simulink model "GHAME_Public"  (R2024a)
settings: Solver=ode8  StartTime=0.0  StopTime=Sim.simulation.duration  FixedStep=0.01  RelTol=1e-3
undefined symbols (not defined in the file): Data, DataPlant, IC, Sim, v0_BE_B
libraries: simulink_extras x8, simulink x1
(part 3 of 3)

== matlab function GHAME_Public/INS/INS/Inertial Navigation System ==
  settings: updateMethod=DISCRETE
  data: muc output; lonc output; latc output; psivdc output; thtvdc output; WBICB output; FSPCB output; dvbec output; SBII input; VBII input; TBI input; WBIB input; FSPB input; ZWG input; ZGPS input; ZST input; delta input; time input; alphacx output; betacx output; altc output; Sim parameter; nzc output; IC parameter; VBECB output; RICI output; EVBI output; ESBI output; MBC output; Data parameter; pdync output; GRAVG output; SBIIC output; VBECD output; TDCI output
function [muc, lonc, latc, psivdc, thtvdc, WBICB, FSPCB, dvbec, ...
    alphacx, betacx, altc, nzc, VBECB, RICI, EVBI, ESBI, MBC, pdync, ...
    GRAVG, SBIIC, VBECD, TDCI] = ins(SBII, VBII, TBI, WBIB, FSPB, ...
    ZWG, ZGPS, ZST, delta, time, Sim, IC, Data)
% INS  Inertial Navigation System model.
%
%   [muc, lonc, latc, psivdc, thtvdc, WBICB, FSPCB, dvbec, alphacx, ...
%       betacx, altc, nzc, VBECB, RICI, EVBI, ESBI, MBC, pdync, cmu, ...
%       c_CBF, dcda, GRAVG] = ins(vmass, SBII, VBII, TBI, WBIB, FSPB, ...
%       ZWG, ZGPS, ZST, delta, time, Sim, IC, Data)
%
%   Navigation states and derived flight quantities from the inertial
%   position, velocity, attitude, body rates and specific force. Based on
%   the CADAC++ 'ins' module of Zipfel, Modeling and Simulation of
%   Aerospace Vehicles.
%
%   Space stabilized INS error model. With Sim.mode.mINS = 1,
%   the tilt, velocity and position errors RICI, EVBI, ESBI are integrated
%   as discrete states with the trapezoidal rule. They start from init_ins
%   and are driven by
%     tilt rate      RICID = TBI' * EWBIB
%     vel err rate   EVBID = TICB*EFSPB - skew(RICI)*TICB*FSPCB + EGRAVI
%     pos err rate   ESBID = EVBI
%   With Sim.mode.mgps > 0 the GPS filter (gps_filter) estimates the
%   position and velocity errors at each GPS update, and they are removed
%   from ESBI and EVBI in the same step. With Sim.mode.mstar > 0 the star
%   tracker (startrack) measures the tilt at each star fix, and it is
%   removed from RICI before the velocity error is computed.
%
%   Onboard aerodynamic model (for rate_observer, with Sim.mode.mrateobs = 1)
%     MBC is the aerodynamic moment as the flight computer would compute
%     it, from the INS altitude, speed, alpha, beta and measured rates, a
%     US 1976 standard atmosphere and the aero tables. No wind is known
%     onboard, so the airspeed is taken as the INS Earth-relative speed.
%     cmu, c_CBF and dcda come from the same tables and are used by the
%     control allocation and the control barrier functions.
%
%   Simulink use (MATLAB Function block)
%     The block contains no random draws. All per run random values come
%     from Sim.ins, built with ins_setup(seed) before each run, and the
%     gyro random walk enters as the unit Gaussian input ZWG from a Random
%     Number block (mean 0, variance 1, sample time dt, seed per run).
%     The GPS Markov noises enter the same way as ZGPS, seed Sim.gps.seed_noise,
%     the star tracker noises as ZST, seed Sim.star.seed_noise.
%     The error states are persistent and reset at every simulation start.
%     The block must run with the discrete sample time dt = Sim.sample_time.
%
%   Inputs
%     vmass    [1x1]  Vehicle mass (kg)
%     SBII     [3x1]  Inertial position (m)
%     VBII     [3x1]  Inertial velocity (m/s)
%     TBI      [3x3]  Body wrt inertial transformation matrix (-)
%     WBIB     [3x1]  Inertial body rates in body axes (rad/s)
%     FSPB     [3x1]  Specific force in body axes (m/s^2)
%     ZWG      [3x1]  Unit Gaussian sample for the gyro random walk (-)
%     ZGPS     [9x1]  Unit Gaussian samples for the GPS Markov noises (-)
%     ZST      [6x1]  Unit Gaussian samples for the star tracker noises (-)
%     delta    [3x1]  Actuator positions [aileron; elevator; rudder] (rad)
%     time     [1x1]  Simulation time (s)
%     Sim      struct Earth model incl. GM, constants, INS mode mINS,
%                     GPS mode mgps, star tracker mode mstar, sample time,
%                     vehicle geometry, INS errors in Sim.ins (see
%                     ins_setup), GPS data in Sim.gps (see gps_setup),
%                     star tracker data in Sim.star (see startrack_setup)
%     IC       struct Earth rotation rate WEII3 (rad/s)
%     Data     struct Aero tables (Data.AeroCoefficients)
%
%   Outputs
%     muc      [1x1]  Aerodynamic roll angle (rad)
%     lonc     [1x1]  Longitude (rad)
%     latc     [1x1]  Geodetic latitude (rad)
%     psivdc   [1x1]  Heading angle (rad)
%     thtvdc   [1x1]  Flight path angle (rad)
%     WBICB    [3x1]  Measured body rates in body axes (rad/s)
%     FSPCB    [3x1]  Measured specific force in body axes (m/s^2)
%     dvbec    [1x1]  Earth-relative speed (m/s)
%     alphacx  [1x1]  Angle of attack (deg)
%     betacx   [1x1]  Angle of sideslip (deg)
%     altc     [1x1]  Altitude (m)
%     nzc      [1x1]  Normal load factor (-)
%     VBECB    [3x1]  Earth-relative velocity in body axes (m/s)
%     RICI     [3x1]  Tilt error (rad)
%     EVBI     [3x1]  Velocity error in inertial axes (m/s)
%     ESBI     [3x1]  Position error in inertial axes (m)
%     MBC      [3x1]  Onboard model of the aerodynamic moment, body axes (Nm)
%     pdync    [1x1]  Onboard dynamic pressure (Pa)
%     cmu      [3x3]  Moment control effectiveness, rows [roll; pitch; yaw],
%                     columns [aileron, elevator, rudder] (m)
%     c_CBF    [9x1]  Control barrier function terms, see cbf_terms
%     dcda     [1x2]  Slopes [dCD/dalpha, dCL/dalpha] (1/rad)
%     GRAVG    [3x1]  Gravitational acceleration, geocentric axes (m/s^2)
%
%   The diagnostics GPSDIAG (see gps_filter) and STDIAG (see startrack) are
%   computed below but are not part of the output list.
%
%   Author:    Thomas Harald Müller
%   GitHub:    https://github.com/ThomasHaraldMueller
%   Copyright: (c) 2026 Thomas Harald Müller, Hamburg, Germany
%   Free to use and modify, provided this notice is kept and the author is credited.

persistent RICI_s EVBI_s ESBI_s RICID EVBID ESBID

%% Constants and configuration
AGRAV    = Sim.earth.AGRAV;             % Standard gravity (m/s^2)
GM       = Sim.earth.GM;                % Earth gravitational constant (m^3/s^2)
GW_CLONG = Sim.earth.GW_CLONG;          % Greenwich longitude at the epoch (rad)
DEG      = Sim.constants.DEG;           % Radian to degree conversion (-)
PI       = Sim.constants.PI;
EPS      = Sim.constants.EPS;
WEII3    = IC.WEII3;                    % Earth rotation rate (rad/s)
mINS     = Sim.mode.mINS;               % INS mode, 0 = ideal INS
dt       = Sim.sample_time;             % Sample time (s)
E        = Sim.ins;                     % Sensor errors and initial error data

%% Error states at simulation start
if isempty(RICI_s)
    [ESBI_s, EVBI_s, RICI_s] = init_ins(mINS, E.frax, E.GAUSS0);
    RICID = zeros(3,1);
    EVBID = zeros(3,1);
    ESBID = zeros(3,1);
end

% GPS filter and star tracker diagnostics, filled in below
GPSDIAG = zeros(6,1);%#ok
STDIAG  = zeros(3,1);%#ok                                                       

%% Navigation solution
if mINS == 0
    % Ideal INS outputs
    TBIC  = TBI;
    FSPCB = FSPB;
    WBICB = WBIB;
    SBIIC = SBII;
    VBIIC = VBII;
else
    % INS derived position, needed for the gravity error
    SBIIC = ESBI_s + SBII;

    % Tilt error from the gyro errors
    [WBICB, EWBIB] = ins_gyro(WBIB, FSPB, ZWG, E, dt);
    RICID_NEW = TBI.' * EWBIB;
    RICI_s = RICI_s + dt/2 * (RICID_NEW + RICID);
    RICID  = RICID_NEW;
    TBIC   = TBI * (eye(3) - skew_sym(RICI_s));

    % Star tracker update of the tilt
    if Sim.mode.mstar > 0
        [URIC, upd_st, STDIAG] = startrack(TBI, TBIC, SBII, ZST, time, Sim); %#ok
        if upd_st
            RICI_s = RICI_s - URIC;
            TBIC   = TBI * (eye(3) - skew_sym(RICI_s));
        end
    end

    % Measured specific force
    EFSPB = ins_accl(FSPB, E);
    FSPCB = E.EWALKA + EFSPB + FSPB;

    % Velocity error from accelerometer, tilt and gravity errors
    EGRAVI    = ins_grav(ESBI_s, SBIIC, norm(SBII), GM);
    TICB      = TBIC.';
    EVBID_NEW = TICB * EFSPB - skew_sym(RICI_s) * TICB * FSPCB + EGRAVI;
    EVBI_s = EVBI_s + dt/2 * (EVBID_NEW + EVBID);
    EVBID  = EVBID_NEW;

    % Position error
    ESBID_NEW = EVBI_s;
    ESBI_s = ESBI_s + dt/2 * (ESBID_NEW + ESBID);
    ESBID  = ESBID_NEW;

    % INS derived position and velocity
    SBIIC = ESBI_s + SBII;
    VBIIC = EVBI_s + VBII;

    % GPS update of the position and velocity errors
    if Sim.mode.mgps > 0
        [SXH, VXH, upd, GPSDIAG] = gps_filter(SBII, VBII, SBIIC, VBIIC, ... 
                                              ZGPS, time, Sim); %#ok
        if upd
            ESBI_s = ESBI_s - SXH;
            EVBI_s = EVBI_s - VXH;
            SBIIC  = ESBI_s + SBII;
            VBIIC  = EVBI_s + VBII;
        end
    end
end

RICI = RICI_s;
EVBI = EVBI_s;
ESBI = ESBI_s;

%% Earth-relative velocity and incidence angles
VEIC  = [-WEII3 * SBIIC(2);
          WEII3 * SBIIC(1);
          0];
VBEIC = VBIIC - VEIC;
VBECB = TBIC * VBEIC;
dvbec = norm(VBECB);

alphac  = atan2(VBECB(3), VBECB(1));
betac   = asin(VBECB(2) / dvbec);
alphacx = alphac * DEG;
betacx  = betac  * DEG;

%% Geodetic position and attitude
[lonc, ~, latc, altc] = cad_geo84_in_cont(time, SBIIC, IC, Sim);
TDCI = cad_tdi84(lonc, latc, time, GW_CLONG, WEII3);

% Heading and flight path angle from the geodetic velocity
VBECD = TDCI * VBEIC;
if VBECD(1) == 0 && VBECD(2) == 0
    psivdc = 0;
    thtvdc = 0;
else
    psivdc = atan2(VBECD(2), VBECD(1));
    thtvdc = atan2(-VBECD(3), hypot(VBECD(1), VBECD(2)));
end

% Geodetic Euler angles
TBD = TBIC * TDCI.';
if abs(TBD(1,3)) < 1
    thtbdc = asin(-TBD(1,3));
    cthtbd = cos(thtbdc);
else
    thtbdc = sgn(-TBD(1,3)) * PI/2;
    cthtbd = EPS;                       % Prevents division by zero at +-90 deg
end
cpsi   = clamp_value(TBD(1,1) / cthtbd, -1, 1);
cphi   = clamp_value(TBD(3,3) / cthtbd, -1, 1);
psibdc = acos(cpsi) * sgn(TBD(1,2));                                        %#ok<NASGU>
phibdc = acos(cphi) * sgn(TBD(2,3));

% Aerodynamic roll angle
num = tan(phibdc) + tan(betac) * ...
      (tan(thtbdc) * cos(alphac) / cos(phibdc) - sin(alphac) / cos(thtbdc));
den = 1 + tan(thtbdc) * sin(alphac) / (cos(betac) * cos(phibdc));
muc = atan2(num, den);

% Normal load factor
nzc = -FSPCB(3) / AGRAV;

%% Air data from the standard atmosphere at the INS altitude
[rhoc, vsoundc] = atmosphere76(altc);
vmachc = dvbec / vsoundc;
pdync  = 0.5 * rhoc * dvbec^2;

GRAVG = cad_grav84(SBIIC, Sim);
%% Onboard aerodynamic model
G = Sim.vehicle.geometry;

% Earth-relative body rates in deg/s, as the aero tables expect them
WBECBx = (WBICB - TBIC * [0; 0; WEII3]) * DEG;

[c_mom] = aero_model(delta * DEG, vmachc, dvbec, alphacx, betacx, ...
                          WBECBx, Data.AeroCoefficients, Sim);
MBC = pdync * G.refa * [G.refb * c_mom(1);
                        G.refc * c_mom(2);
                        G.refb * c_mom(3)];
end


%% Local functions, INS sensor and error models =========================

function [WBICB, EWBIB] = ins_gyro(WBIB, FSPB, ZWG, E, dt)
% INS_GYRO  Gyro measured body rates and their error, with misalignment,
%   scale factor, bias, mass unbalance and random walk.

% Misalignment and scale factor plus bias
EGB   = diag(E.ESCALG) + skew_sym(E.EMISG);
EMSBG = E.EBIASG + EGB * WBIB;

% Spin axis sensitivity (mass unbalance)
EUG = E.EUNBG .* FSPB;

% Random walk, white noise with intensity EWALKG
EWG = E.EWALKG / sqrt(dt) * ZWG;

% Total error and measured body rates
EWBIB = EMSBG + EUG + EWG;
WBICB = WBIB + EWBIB;
end


function EFSPB = ins_accl(FSPB, E)
% INS_ACCL  Accelerometer error with misalignment, scale factor and bias.

EAB   = diag(E.ESCALA) + skew_sym(E.EMISA);
EFSPB = E.EBIASA + EAB * FSPB;
end


function EGRAVI = ins_grav(ESBI, SBIIC, dbi, GM)
% INS_GRAV  First order gravitational acceleration error (Zipfel, Eq. 10.94).

dbic   = norm(SBIIC);
ed     = dbic - dbi;
dum    = GM / dbic^3;
EGRAVI = -dum * ESBI - 3 * dum * ed / dbic * SBIIC;
end


%% Local functions, onboard aerodynamic model ===========================

function [alpha_vec, mach_vec, dalpha_deg] = aero_grid()
% AERO_GRID  Breakpoints of the aero tables and the step used for the
%   central differences in alpha.
%
%     alpha_vec   Angle of attack breakpoints (deg)
%     mach_vec    Mach number breakpoints (-)
%     dalpha_deg  Step of the central difference in alpha (deg)

alpha_vec  = (-3:3:+21);
mach_vec   = [0.4 0.6 0.8 0.9 0.95 1.05 1.2 1.5 2.0 3.0 6.0 12.0 24.0];
dalpha_deg = 1.0;
end


function c_mom = aero_model(deltax, vmach, DVBA, alphax, betax, WBEBx, Tab, Sim)
% AERO_MODEL  Onboard body-axis moment coefficients [Cl; Cm; Cn] and the
%   moment control effectiveness. Same tables and units as the plant
%   aerodynamics function, angles and deflections in deg, rates in deg/s.

RAD  = Sim.constants.RAD;
refb = Sim.vehicle.geometry.refb;
refc = Sim.vehicle.geometry.refc;
[alpha_vec, mach_vec] = aero_grid();

% Table lookup, clamped to the table range
vm = clamp_value(vmach,  mach_vec(1),  mach_vec(end));
al = clamp_value(alphax, alpha_vec(1), alpha_vec(end));
lk = @(table) interp2(mach_vec, alpha_vec, table, vm, al, 'linear');

% Nondimensional rates p*b/(2V), q*c/(2V), r*b/(2V)
pn = WBEBx(1) * RAD * refb / (2 * DVBA);
qn = WBEBx(2) * RAD * refc / (2 * DVBA);
rn = WBEBx(3) * RAD * refb / (2 * DVBA);

% Rolling, pitching and yawing moment
cll = lk(Tab.CLLB_tab) * betax + lk(Tab.CLLDA_tab) * deltax(1) + ...
      lk(Tab.CLLDR_tab) * deltax(3) + lk(Tab.CLLP_tab) * pn + lk(Tab.CLLR_tab) * rn;
clm = lk(Tab.CM0_tab) + lk(Tab.CMA_tab) * alphax + lk(Tab.CMDE_tab) * deltax(2) + ...
      lk(Tab.CMQ_tab) * qn;
cln = lk(Tab.CNB_tab) * betax + lk(Tab.CNDA_tab) * deltax(1) + ...
      lk(Tab.CNDR_tab) * deltax(3) + lk(Tab.CNP_tab) * pn + lk(Tab.CNR_tab) * rn;
c_mom = [cll; clm; cln];

end


%% Local functions, GPS =================================================

function [SXH, VXH, upd, GPSDIAG] = gps_filter(SBII, VBII, SBIIC, VBIIC, ZGPS, time, Sim)
% GPS_FILTER  GPS receiver and extended Kalman filter for INS aiding.
%
%   [SXH, VXH, upd, GPSDIAG] = gps_filter(SBII, VBII, SBIIC, VBIIC, ...
%       ZGPS, time, Sim)
%
%   Port of the CADAC++ 'gps' module of Zipfel, Modeling and Simulation of
%   Aerospace Vehicles. Four pseudo-ranges and four range rates are measured
%   from the four GPS satellites (quadriga) with the lowest GDOP. An 8 state
%   error filter (3 position, 3 velocity, user clock bias and frequency)
%   estimates the INS position and velocity errors at every GPS update.
%   The caller (ins) subtracts SXH and VXH from its error states when
%   upd = 1. The filter state is reset to zero after each update.
%
%   GPS is used in a run with Sim.mode.mgps = 1. Signal acquisition takes
%   Sim.gps.gps_acqtime before the first update. Internal GPS mode
%     0  no GPS
%     1  initialize filter, start signal acquisition
%     2  filter extrapolation between updates
%     3  update epoch, measurement and filter correction
%
%   Measurement errors are pseudo-range biases (constant per run), first
%   order Markov noise on pseudo-ranges, range rates and user clock
%   frequency, and the user clock bias obtained by integrating the clock
%   frequency error. The Markov processes are driven by the unit Gaussian
%   input ZGPS, which comes from a Random Number block in Simulink.
%
%   Inputs
%     SBII     [3x1]  True inertial position (m)
%     VBII     [3x1]  True inertial velocity (m/s)
%     SBIIC    [3x1]  INS inertial position (m)
%     VBIIC    [3x1]  INS inertial velocity (m/s)
%     ZGPS     [9x1]  Unit Gaussian samples for the Markov noises,
%                     [pseudo-range 1-4; range rate 1-4; clock frequency] (-)
%     time     [1x1]  Simulation time (s)
%     Sim      struct Earth model, sample time, GPS mode, GPS data in Sim.gps
%
%   Outputs
%     SXH      [3x1]  Estimated INS position error, inertial axes (m)
%     VXH      [3x1]  Estimated INS velocity error, inertial axes (m/s)
%     upd      [1x1]  1 at an update epoch, else 0 (-)
%     GPSDIAG  [6x1]  [std pos (m); std vel (m/s); std clock bias (m);
%                      GDOP (-); GPS mode (-); update flag (-)]
%
%   Author:    Thomas Harald Müller
%   GitHub:    https://github.com/ThomasHaraldMueller
%   Copyright: (c) 2026 Thomas Harald Müller, Hamburg, Germany
%   Free to use and modify, provided this notice is kept and the author is credited.

persistent mgps PP QQ RR PHI gps_epoch gps_acq ucbias_error ucfreqm XM gdop
persistent SV rsi wsi incl

G  = Sim.gps;
dt = Sim.sample_time;

% Initialization at simulation start
if isempty(mgps)
    mgps         = Sim.mode.mgps;       % 0: without GPS, 1: with GPS
    PP           = zeros(8);
    QQ           = zeros(8);
    RR           = zeros(8);
    PHI          = eye(8);
    gps_epoch    = 0;
    gps_acq      = 0;
    ucbias_error = G.ucbias0;           % User clock bias error (m)
    ucfreqm      = 0;                   % Clock frequency error, last step (m/s)
    XM           = G.markov0;           % Markov states [pr 1-4; dr 1-4; ucfreq]
    gdop         = 0;
    [SV, rsi, wsi, incl] = gps_sv_init(Sim.earth.GM);
end

SXH = zeros(3,1);
VXH = zeros(3,1);
upd = 0;

% First order Markov noises, exact discretization
a  = exp(-dt ./ G.tau_markov);
XM = a .* XM + G.sig_markov .* sqrt(1 - a.^2) .* ZGPS;
pr_noise     = XM(1:4);                 % Pseudo-range noise (m)
dr_noise     = XM(5:8);                 % Range rate noise (m/s)
ucfreq_error = XM(9);                   % User clock frequency error (m/s)

% Filter initialization, also used to re-acquire after a loss of satellites
if mgps == 1
    fp = 1 + G.factp;
    fq = 1 + G.factq;
    fr = 1 + G.factr;
    PP = diag(([G.ppos*[1 1 1], G.pvel*[1 1 1], G.pclockb, G.pclockf] * fp).^2);
    QQ = diag(([G.qpos*[1 1 1], G.qvel*[1 1 1], G.qclockb, G.qclockf] * fq).^2);
    RR = diag(([G.rpos*[1 1 1 1], G.rvel*[1 1 1 1]] * fr).^2);

    % Error dynamics and state transition matrix, constant
    FF = zeros(8);
    FF(1,4) = 1;
    FF(2,5) = 1;
    FF(3,6) = 1;
    FF(7,8) = 1;
    FF(8,8) = -1 / G.uctime_cor;
    PHI = eye(8) + FF * dt + FF * FF * (dt^2 / 2);

    gps_acq   = 1;
    gps_epoch = time;
    mgps      = 2;
end

% Clock error growth and covariance extrapolation
if mgps == 2
    if gps_acq
        dtime_gps = G.gps_acqtime;      % Signal acquisition delay (s)
    else
        dtime_gps = G.gps_step;         % Update interval (s)
    end
    if time - gps_epoch >= dtime_gps - 1e-9
        mgps = 3;
    end

    % User clock bias from the frequency error, trapezoidal integration
    ucbias_error = ucbias_error + (ucfreq_error + ucfreqm) * dt/2;
    ucfreqm      = ucfreq_error;

    PP = PHI * (PP + QQ * dt/2) * PHI.' + QQ * dt/2;
end

% Update epoch
if mgps == 3
    gps_acq   = 0;
    gps_epoch = time;
    [SSQ, VSQ, gdop_q, nvis] = gps_quadriga(SV, rsi, wsi, incl, ...
        G.almanac_time, G.del_rearth, Sim.earth.REARTH, time, SBII);

    if nvis < 4
        % Not enough satellites visible, re-acquire
        mgps = 1;
    else
        gdop = gdop_q;
        ZZ = zeros(8,1);
        HH = zeros(8,8);
        for i = 1:4
            SSII = SSQ(:,i);
            VSII = VSQ(:,i);

            % True and measured pseudo-range and range rate
            SSBI      = SSII - SBII;
            dsb       = norm(SSBI);
            USSBI     = SSBI / dsb;
            dsb_meas  = dsb + G.pr_bias(i) + pr_noise(i) + ucbias_error;
            dvsb      = (VSII - VBII).' * USSBI;
            dvsb_meas = dvsb + dr_noise(i) + ucfreq_error;

            % INS derived pseudo-range and range rate
            SSBIC = SSII - SBIIC;
            dsbc  = norm(SSBIC);
            dvsbc = (VSII - VBIIC).' * SSBIC / dsbc;

            % Measurement residuals and observation matrix
            ZZ(i)       = dsb_meas  - dsbc;
            ZZ(i+4)     = dvsb_meas - dvsbc;
            HH(i,1:3)   = USSBI.';
            HH(i,7)     = 1;
            HH(i+4,4:6) = USSBI.';      % Range rate residual in m/s, no
            HH(i+4,8)   = 1;            % gps_step factor (C++ used one)
        end

        % Kalman gain, state and covariance correction
        KK = (PP * HH.') / (HH * PP * HH.' + RR);
        XH = KK * ZZ;
        PP = (eye(8) - KK * HH) * PP;
        PP = (PP + PP.') / 2;

        % User clock bias correction
        ucbias_error = ucbias_error - XH(7);

        % Estimated INS errors, handed to ins
        SXH  = XH(1:3);
        VXH  = XH(4:6);
        upd  = 1;
        mgps = 2;
    end
end

GPSDIAG = [sqrt(PP(1,1)); sqrt(PP(4,4)); sqrt(PP(7,7)); gdop; mgps; upd];
end


function [SSQ, VSQ, gdop, nvis] = gps_quadriga(SV, rsi, wsi, incl, almanac_time, del_rearth, REARTH, time, SBII)
% GPS_QUADRIGA  Visible GPS satellites and the four with the lowest GDOP.
%   Circular orbits, 6 planes at 60 deg right ascension spacing, 55 deg
%   inclination. Returns their inertial positions and velocities as
%   columns, nvis < 4 means no valid quadriga.

% Satellite positions and velocities, argument of latitude propagated in time
Om  = SV(:,1);
u   = SV(:,2) + (almanac_time + time) * wsi;
si  = sin(incl);
ci  = cos(incl);
vel = rsi * wsi;

SSII = rsi * [ (cos(Om).*cos(u) - sin(Om).*sin(u)*ci).';
               (sin(Om).*cos(u) + cos(Om).*sin(u)*ci).';
               (sin(u)*si).' ];
VSII = vel * [ (-cos(Om).*sin(u) - sin(Om).*cos(u)*ci).';
               (-sin(Om).*sin(u) + cos(Om).*cos(u)*ci).';
               (cos(u)*si).' ];

% Visibility, inside the cone of the satellite or high enough for line of sight
dbi     = norm(SBII);
rclear  = REARTH + del_rearth;          % Radius for clear signal reception (m)
epsilon = acos(rclear / rsi);           % Grazing angle at the Earth center (rad)

vis  = zeros(24,1);
nvis = 0;
for i = 1:24
    cdel  = SSII(:,i).' * SBII / (rsi * dbi);
    delta = acos(clamp_value(cdel, -1, 1));
    rmin  = rclear / cos(delta - epsilon);
    if delta < epsilon || (rmin > 0 && rmin < dbi)
        nvis = nvis + 1;
        vis(nvis) = i;
    end
end

SSQ  = zeros(3,4);
VSQ  = zeros(3,4);
gdop = 1e10;
if nvis < 4
    return;
end

% Quadriga with the lowest GDOP among all combinations of visible satellites
quad = vis(1:4);
for i1 = 1:nvis-3
    for i2 = i1+1:nvis-2
        for i3 = i2+1:nvis-1
            for i4 = i3+1:nvis
                s = [vis(i1); vis(i2); vis(i3); vis(i4)];
                HGPS = ones(4,4);
                for m = 1:4
                    d = SBII - SSII(:,s(m));
                    HGPS(m,1:3) = d.' / norm(d);
                end
                M = HGPS * HGPS.';
                if rcond(M) > 1e-12
                    gdop_local = sqrt(trace(inv(M)));
                    if gdop_local < gdop
                        gdop = gdop_local;
                        quad = s;
                    end
                end
            end
        end
    end
end

SSQ = SSII(:,quad);
VSQ = VSII(:,quad);
end


function [SV, rsi, wsi, incl] = gps_sv_init(GM)
% GPS_SV_INIT  GPS constellation from the week 224 almanac (2003),
%   reduced to circular orbits. Rows are slots 1-24, planes A-F with four
%   satellites each, [right ascension (rad), argument of latitude (rad)].

SV = [ 0.9947,  1.0371;   % A plane
       0.9947,  2.7284;
       0.9947, -2.9855;
       0.9947, -0.9112;
       1.9197,  1.6417;   % B plane
       1.9197, -2.2572;
       1.9197, -0.7270;
       1.9197, -0.1626;
       2.9668,  0.5080;   % C plane
       2.9668,  2.1743;
       2.9668,  2.7649;
       2.9668, -1.8197;
       4.0140,  0.9408;   % D plane
       4.0140,  2.4279;
       4.0140, -3.1153;
       4.0140, -0.7710;
       5.0611,  1.3270;   % E plane
       5.0611,  2.1057;
       5.0611, -2.5338;
       5.0611, -0.2883;
       6.1082,  0.3998;   % F plane
       6.1082,  2.3427;
       6.1082, -1.8972;
       6.1082, -1.4035 ];

rsi  = 26560000;                        % Orbit radius (m)
wsi  = sqrt(GM / rsi^3);                % Orbital rate, half a sidereal day (rad/s)
incl = 0.95986;                         % Inclination, 55 deg (rad)
end


%% Local functions, star tracker ========================================

function [URIC, upd, STDIAG] = startrack(TBI, TBIC, SBII, ZST, time, Sim)
% STARTRACK  Star tracker for INS tilt correction.
%
%   [URIC, upd, STDIAG] = startrack(TBI, TBIC, SBII, ZST, time, Sim)
%
%   Port of the CADAC++ 'startrack' module of Zipfel, Modeling and
%   Simulation of Aerospace Vehicles. From a catalog of 25 bright stars the
%   visible ones are selected and the three with the largest parallelepiped
%   volume (triad) are tracked. Each star direction is measured in body
%   axes with the true attitude, corrupted by tracker bias and noise, and
%   converted back to inertial axes with the INS attitude TBIC. Comparing
%   measured and true directions gives I + skew(RICI), from which the INS
%   tilt is read directly. The caller (ins) subtracts URIC from RICI when
%   upd = 1. There is no filter, every fix replaces the tilt estimate.
%
%   The star tracker is used in a run with Sim.mode.mstar = 1. It works only
%   above Sim.star.startrack_alt, acquisition takes Sim.star.star_acqtime
%   before the first fix. Internal mode
%     0  no star tracker
%     1  initialized, waiting for the minimum altitude
%     2  waiting for the next fix
%     3  star fix and tilt correction
%
%   Inputs
%     TBI      [3x3]  True body wrt inertial transformation matrix (-)
%     TBIC     [3x3]  INS body wrt inertial transformation matrix (-)
%     SBII     [3x1]  True inertial position (m)
%     ZST      [6x1]  Unit Gaussian samples for the Markov noises,
%                     [azimuth 1-3; elevation 1-3] (-)
%     time     [1x1]  Simulation time (s)
%     Sim      struct Earth model, sample time, star tracker mode, data in
%                     Sim.star (see startrack_setup)
%
%   Outputs
%     URIC     [3x1]  Measured INS tilt, inertial axes (rad)
%     upd      [1x1]  1 at a star fix, else 0 (-)
%     STDIAG   [3x1]  [triad volume (-); star tracker mode (-); update flag (-)]
%
%   Author:    Thomas Harald Müller
%   GitHub:    https://github.com/ThomasHaraldMueller
%   Copyright: (c) 2026 Thomas Harald Müller, Hamburg, Germany
%   Free to use and modify, provided this notice is kept and the author is credited.

persistent mstar starfix_epoch star_acq XM star_volume

S  = Sim.star;
dt = Sim.sample_time;

% Initialization at simulation start
if isempty(mstar)
    mstar         = Sim.mode.mstar;     % 0: without star tracker, 1: with
    starfix_epoch = 0;
    star_acq      = 0;
    XM            = S.markov0;          % Markov states [az 1-3; el 1-3]
    star_volume   = 0;
end

URIC = zeros(3,1);
upd  = 0;

% First order Markov noises, exact discretization
a  = exp(-dt ./ S.tau_markov);
XM = a .* XM + S.sig_markov .* sqrt(1 - a.^2) .* ZST;

% Altitude over the mean Earth radius, only used for the availability check
alt = norm(SBII) - Sim.earth.REARTH;

% Initialization, acquisition starts once above the dense atmosphere
if mstar == 1
    star_acq      = 1;
    starfix_epoch = time;
    if alt > S.startrack_alt
        mstar = 2;
    end
end

% Delay before the first fix and between fixes
if mstar == 2
    if star_acq
        dtime_star = S.star_acqtime;    % Initial acquisition delay (s)
    else
        dtime_star = S.star_step;       % Fix interval (s)
    end
    if time - starfix_epoch >= dtime_star - 1e-9 && alt > S.startrack_alt
        mstar = 3;
    end
end

% Star fix
if mstar == 3
    star_acq      = 0;
    starfix_epoch = time;
    mstar         = 2;
    [UTRIAD, vol, nvis] = star_triad(star_catalog(), S.star_el_min * pi/180, SBII);

    if nvis >= 3
        star_volume = vol;
        TRIAD_MEAS  = zeros(3,3);
        for i = 1:3
            % True direction in body axes, azimuth and elevation
            USIB = TBI * UTRIAD(:,i);
            az   = atan2(USIB(2), USIB(1));
            el   = atan2(-USIB(3), hypot(USIB(1), USIB(2)));

            % Measurement with tracker bias and noise
            az_m  = az + S.az_bias(i) + XM(i);
            el_m  = el + S.el_bias(i) + XM(i+3);
            USIBM = [cos(el_m) * cos(az_m);
                     cos(el_m) * sin(az_m);
                    -sin(el_m)];

            % Back to inertial axes with the INS attitude, the tilt enters here
            TRIAD_MEAS(:,i) = TBIC.' * USIBM;
        end

        % RDIFF = I + skew(RICI), tilt from its skew symmetric part
        RDIFF = TRIAD_MEAS / UTRIAD;
        URIC  = [RDIFF(3,2) - RDIFF(2,3);
                 RDIFF(1,3) - RDIFF(3,1);
                 RDIFF(2,1) - RDIFF(1,2)] / 2;
        upd   = 1;
    end
end

STDIAG = [star_volume; mstar; upd];
end


function [UTRIAD, star_volume, nvis] = star_triad(STARS, el_min, SBII)
% STAR_TRIAD  Visible stars and the three with the largest parallelepiped
%   volume. Returns their inertial unit vectors as columns, nvis < 3 means
%   no valid triad.

UBII = SBII / norm(SBII);
vis  = zeros(25,1);
nvis = 0;
for i = 1:25
    % Star elevation over the local horizontal, star at infinity
    elstar = asin(clamp_value(STARS(:,i).' * UBII, -1, 1));
    if elstar > el_min
        nvis = nvis + 1;
        vis(nvis) = i;
    end
end

UTRIAD      = eye(3);
star_volume = 0;
if nvis < 3
    return;
end

triad = vis(1:3);
for i1 = 1:nvis-2
    for i2 = i1+1:nvis-1
        for i3 = i2+1:nvis
            vol = abs(STARS(:,vis(i1)).' * cross(STARS(:,vis(i2)), STARS(:,vis(i3))));
            if vol > star_volume
                star_volume = vol;
                triad = [vis(i1); vis(i2); vis(i3)];
            end
        end
    end
end

UTRIAD = STARS(:,triad);
end


function STARS = star_catalog()
% STAR_CATALOG  25 bright stars, unit vectors in J2000 as columns.
%   1 Sirius, 2 Canopus, 3 Rigil Kent, 4 Arcturus, 5 Vega, 6 Rigel,
%   7 Capella, 8 Procyon, 9 Achernar, 10 Hadar, 11 Altair, 12 Aldebaran,
%   13 Acrux, 14 Betelgeuse, 15 Antares, 16 Spica, 17 Pollux,
%   18 Fomalhaut, 19 Deneb, 20 Mimosa, 21 Regulus, 22 Adhara,
%   23 Bellatrix, 24 Shaula, 25 El Nath

STARS = [ -.179457,  .947482, -.264715;
          -.062053,  .621699, -.780794;
          -.395709, -.321011, -.860446;
          -.787739, -.518432,  .332710;
           .119339, -.770884,  .625697;
           .205167,  .969392, -.134851;
           .141589,  .680716,  .718733;
          -.407741,  .908325,  .093239;
           .504096,  .224174, -.834046;
          -.434428, -.251576, -.864859;
           .449879, -.880088,  .151836;
           .355451,  .890944,  .282620;
          -.479412, -.049965, -.876167;
           .032446,  .991140,  .128796;
          -.357911, -.827083, -.433397;
          -.923975, -.348220, -.158158;
          -.380630,  .795326,  .471781;
           .846646, -.247176, -.471268;
           .453017, -.541322,  .708340;
          -.511331, -.101246, -.853399;
          -.858250,  .467448,  .211893;
          -.217999,  .863108, -.455545;
           .161912,  .980685,  .109734;
          -.103643, -.792588, -.600885;
           .140796,  .866902,  .478181 ].';
end


%% Local functions, Earth model and atmosphere ==========================

function [lon, lon_cel, lat, alt] = cad_geo84_in_cont(time, SBII, IC, Sim)
% CAD_GEO84_IN_CONT  Inertial position to geodetic longitude, latitude and
%   altitude on the WGS84 ellipsoid.
%
%   [lon, lon_cel, lat, alt] = cad_geo84_in_cont(time, SBII, IC, Sim)
%
%   Latitude and altitude use Bowring's closed-form method, which is
%   accurate to well below a millimetre for altitudes up to orbital heights.
%
%   Inputs
%     time   [1x1]  Simulation time since the initial epoch (s)
%     SBII   [3x1]  Position in inertial coordinates (m)
%     IC     struct Earth rotation rate (IC.WEII3, rad/s)
%     Sim    struct Ellipsoid parameters (flattening, semi-major axis) and
%                   Greenwich longitude at the initial epoch (rad)
%
%   Outputs
%     lon      [1x1]  Geodetic longitude in (-pi, pi] (rad)
%     lon_cel  [1x1]  Celestial longitude, measured in the inertial frame (rad)
%     lat      [1x1]  Geodetic latitude (rad)
%     alt      [1x1]  Altitude above the ellipsoid (m)
%
%   Author:    Thomas Harald Müller
%   GitHub:    https://github.com/ThomasHaraldMueller
%   Copyright: (c) 2026 Thomas Harald Müller, Hamburg, Germany
%   Free to use and modify, provided this notice is kept and the author is credited.

% Ellipsoid and Earth rotation
f        = Sim.earth.FLATTENING;
a        = Sim.earth.SMAJOR_AXIS;
GW_CLONG = Sim.earth.GW_CLONG;
WEII3    = IC.WEII3;

b   = a * (1 - f);              % Semi-minor axis
e2  = 2*f - f^2;                % First eccentricity squared
ep2 = e2 / (1 - e2);            % Second eccentricity squared

x = SBII(1);
y = SBII(2);
z = SBII(3);

% Longitude, inertial longitude minus the Earth rotation since the epoch
lon_cel = atan2(y, x);
lon     = lon_cel - WEII3 * time - GW_CLONG;
lon     = atan2(sin(lon), cos(lon));            % Wrap to (-pi, pi]

% Latitude (Bowring)
p   = sqrt(x^2 + y^2);                          % Distance from the polar axis
u   = atan2(z * a, p * b);                      % Parametric latitude
lat = atan2(z + ep2 * b * sin(u)^3, ...
            p - e2  * a * cos(u)^3);

% Altitude, form valid at all latitudes, including the poles where
% p/cos(lat) is singular
N   = a / sqrt(1 - e2 * sin(lat)^2);            % Prime vertical radius of curvature
alt = p * cos(lat) + z * sin(lat) - a^2 / N;
end


function TDI = cad_tdi84(lon, lat, time, GW_CLONG, WEII3)
% CAD_TDI84  Geodetic wrt inertial transformation matrix.

lon_cel = GW_CLONG + WEII3 * time + lon;    % Celestial longitude
slat = sin(lat);
clat = cos(lat);
slon = sin(lon_cel);
clon = cos(lon_cel);

TDI = [-slat * clon, -slat * slon,  clat;
       -slon,         clon,         0;
       -clat * clon, -clat * slon, -slat];
end


function GRAVG = cad_grav84(SBII, Sim)
% CAD_GRAV84  Gravitational acceleration with J2 in geocentric coordinates.
%
%   GRAVG = cad_grav84(SBII, Sim)
%
%   Uses the normalized second zonal harmonic C20 of the WGS84 field.
%   The geocentric frame G is north, east, down with the down axis pointing
%   to the Earth centre. The east component is zero for a zonal field.
%
%   Inputs
%     SBII    [3x1]  Position in inertial coordinates (m)
%     Sim     struct Earth constants (GM, semi-major axis, normalized C20 < 0)
%
%   Output
%     GRAVG   [3x1]  Gravitational acceleration in geocentric axes (m/s^2)
%
%   Author:    Thomas Harald Müller
%   GitHub:    https://github.com/ThomasHaraldMueller
%   Copyright: (c) 2026 Thomas Harald Müller, Hamburg, Germany
%   Free to use and modify, provided this notice is kept and the author is credited.

GM  = Sim.earth.GM;
a   = Sim.earth.SMAJOR_AXIS;
C20 = Sim.earth.C20;

r    = norm(SBII);
latc = asin(SBII(3) / r);           % Geocentric latitude
slat = sin(latc);
clat = cos(latc);

g0 = GM / r^2;                      % Point-mass gravity
k  = sqrt(5) * C20 * (a / r)^2;     % J2 scaling, negative for C20 < 0

% Gradient of V = GM/r * (1 + C20*(a/r)^2 * sqrt(5)/2 * (3*sin(lat)^2 - 1))
GRAVG = [ 3 * g0 * k * slat * clat;                 % North (towards equator)
          0;                                        % East
          g0 * (1 + 1.5 * k * (3 * slat^2 - 1)) ];  % Down
end


function [rho, vsound] = atmosphere76(alt)
% ATMOSPHERE76  US 1976 standard atmosphere up to 86 km, density (kg/m^3)
%   and speed of sound (m/s) from the geometric altitude (m).

R  = 287.05287;                         % Gas constant of air (J/kg/K)
g0 = 9.80665;                           % Standard gravity (m/s^2)
r0 = 6356766;                           % Earth radius for geopotential altitude (m)
HB = [0, 11000, 20000, 32000, 47000, 51000, 71000, 84852];   % Layer bases (m)
LB = [-6.5e-3, 0, 1e-3, 2.8e-3, 0, -2.8e-3, -2e-3];          % Lapse rates (K/m)

h = r0 * alt / (r0 + alt);              % Geopotential altitude (m)
h = clamp_value(h, 0, HB(end));

T = 288.15;
P = 101325;
for i = 1:7
    dh = min(h, HB(i+1)) - HB(i);
    if dh <= 0
        break;
    end
    if LB(i) == 0
        P = P * exp(-g0 * dh / (R * T));
    else
        Tn = T + LB(i) * dh;
        P  = P * (Tn / T)^(-g0 / (R * LB(i)));
        T  = Tn;
    end
end

rho    = P / (R * T);
vsound = sqrt(1.4 * R * T);
end


%% Local functions, utilities ===========================================

function S = skew_sym(v)
% SKEW_SYM  Skew symmetric matrix, S*x = cross(v, x).

S = [ 0    -v(3)  v(2);
      v(3)  0    -v(1);
     -v(2)  v(1)  0   ];
end


function s = sgn(x)
% SGN  Sign function returning +1 for x >= 0, as in CADAC.

s = 1 - 2*(x < 0);
end


function value_clamped = clamp_value(value, min_value, max_value)
% CLAMP_VALUE  Saturate value to [min_value, max_value].

value_clamped = max(min(value, max_value), min_value);
end

== matlab function GHAME_Public/GHAME Airframe/Dynamics/NEWTON/Geodetic position update/Geodetic Position ==
  data: lon output; lon_cel output; time input; SBII input; IC parameter; lat output; alt output; Sim parameter
function [lon, lon_cel, lat, alt] = cad_geo84_in_cont(time, SBII, IC, Sim)
% CAD_GEO84_IN_CONT  Inertial position to geodetic longitude, latitude and
%   altitude on the WGS84 ellipsoid.
%
%   [lon, lon_cel, lat, alt] = cad_geo84_in_cont(time, SBII, IC, Sim)
%
%   Latitude and altitude use Bowring's closed-form method, which is
%   accurate to well below a millimetre for altitudes up to orbital heights.
%
%   Inputs
%     time   [1x1]  Simulation time since the initial epoch (s)
%     SBII   [3x1]  Position in inertial coordinates (m)
%     IC     struct Earth rotation rate (IC.WEII3, rad/s)
%     Sim    struct Ellipsoid parameters (flattening, semi-major axis) and
%                   Greenwich longitude at the initial epoch (rad)
%
%   Outputs
%     lon      [1x1]  Geodetic longitude in (-pi, pi] (rad)
%     lon_cel  [1x1]  Celestial longitude, measured in the inertial frame (rad)
%     lat      [1x1]  Geodetic latitude (rad)
%     alt      [1x1]  Altitude above the ellipsoid (m)

%   Author:    Thomas Harald Müller
%   GitHub:    https://github.com/ThomasHaraldMueller
%   Copyright: (c) 2026 Thomas Harald Müller, Hamburg, Germany
%   Free to use and modify, provided this notice is kept and the author is credited.

%% Ellipsoid and Earth rotation
f     = Sim.earth.FLATTENING;
a     = Sim.earth.SMAJOR_AXIS;
GW_CLONG = Sim.earth.GW_CLONG;
WEII3 = IC.WEII3;

b   = a * (1 - f);              % Semi-minor axis
e2  = 2*f - f^2;                % First eccentricity squared
ep2 = e2 / (1 - e2);            % Second eccentricity squared

x = SBII(1);
y = SBII(2);
z = SBII(3);

%% Longitude
% Inertial longitude minus the Earth rotation since the epoch
lon_cel = atan2(y, x);
lon     = lon_cel - WEII3 * time - GW_CLONG;
lon     = atan2(sin(lon), cos(lon));            % Wrap to (-pi, pi]

%% Latitude (Bowring)
p = sqrt(x^2 + y^2);                            % Distance from the polar axis
u = atan2(z * a, p * b);                        % Parametric latitude

lat = atan2(z + ep2 * b * sin(u)^3, ...
            p - e2  * a * cos(u)^3);

%% Altitude
% Form valid at all latitudes, including the poles where p/cos(lat) is singular
N   = a / sqrt(1 - e2 * sin(lat)^2);            % Prime vertical radius of curvature
alt = p * cos(lat) + z * sin(lat) - a^2 / N;

end

== matlab function GHAME_Public/GHAME Airframe/Dynamics/NEWTON/Geodetic position update/TM Inertial to Geocentric ==
  data: TDI input; lat input; alt input; TGI output; TDI output; lat output; Sim parameter; alt output
function [TGI, TDI, lat, alt] = cad_tgi84(TDI, lat, alt, Sim)
% CAD_TGI84  Transformation matrix from inertial to geocentric coordinates.
%
%   [TGI, TDI, lat, alt] = cad_tgi84(TDI, lat, alt, Sim)
%
%   The geocentric frame G is the geodetic frame D rotated about its east
%   axis by the deflection dd between the ellipsoid normal and the radius
%   vector, so that its down axis points to the Earth centre. dd and the
%   ellipsoid radius r0 use series expansions in the flattening, accurate
%   to about 1e-5 rad and 0.1 m below 100 km altitude.
%
%   Inputs
%     TDI   [3x3]  Transformation matrix [T]^DI, inertial to geodetic
%     lat   [1x1]  Geodetic latitude (rad)
%     alt   [1x1]  Altitude above the ellipsoid (m)
%     Sim   struct Ellipsoid parameters (flattening, semi-major axis)
%
%   Outputs
%     TGI   [3x3]  Transformation matrix [T]^GI, inertial to geocentric
%     TDI, lat, alt  Passed through unchanged

%   Author:    Thomas Harald Müller
%   GitHub:    https://github.com/ThomasHaraldMueller
%   Copyright: (c) 2026 Thomas Harald Müller, Hamburg, Germany
%   Free to use and modify, provided this notice is kept and the author is credited.

f = Sim.earth.FLATTENING;
a = Sim.earth.SMAJOR_AXIS;

% Ellipsoid radius at the given geodetic latitude
r0 = a * (1 - f*(1 - cos(2*lat))/2 + 5*f^2*(1 - cos(4*lat))/16);

% Deflection between geodetic and geocentric vertical, decreasing with altitude
dd = f * sin(2*lat) * (1 - f/2 - alt/r0);

% Rotation about the east axis from geodetic to geocentric
TGD = [cos(dd), 0, -sin(dd);
       0,       1,  0;
       sin(dd), 0,  cos(dd)];

TGI = TGD * TDI;

end

== matlab function GHAME_Public/GHAME Airframe/Dynamics/NEWTON/Geodetic position update/TM Inertial to Geodetic ==
  data: lon_cel input; TDI output; lat input; lat output
function [TDI, lat] = cad_tdi84(lon_cel, lat)
% CAD_TDI84  Transformation matrix from inertial to geodetic coordinates.
%
%   [TDI, lat] = cad_tdi84(lon_cel, lat)
%
%   The geodetic frame D is north, east, down at the vehicle position.
%   Using the celestial longitude makes the matrix account for Earth
%   rotation directly, so no time or rotation rate is needed here.
%
%   Inputs
%     lon_cel  [1x1]  Celestial longitude, measured in the inertial frame (rad)
%     lat      [1x1]  Geodetic latitude (rad)
%
%   Outputs
%     TDI      [3x3]  Transformation matrix [T]^DI, so that v_D = TDI * v_I
%     lat      [1x1]  Geodetic latitude, passed through unchanged

%   Author:    Thomas Harald Müller
%   GitHub:    https://github.com/ThomasHaraldMueller
%   Copyright: (c) 2026 Thomas Harald Müller, Hamburg, Germany
%   Free to use and modify, provided this notice is kept and the author is credited.

slat = sin(lat);
clat = cos(lat);
slon = sin(lon_cel);
clon = cos(lon_cel);

TDI = [ -slat*clon,  -slat*slon,   clat;     % North
        -slon,        clon,        0;        % East
        -clat*clon,  -clat*slon,  -slat ];   % Down

end

== matlab function GHAME_Public/GHAME Airframe/Forces and Moments/FORCE/Aerodynamic moments ==
  data: c_moment input; pdynmc input; FMB output; Sim parameter
function FMB = computeMoment(c_moment, pdynmc, Sim)
% COMPUTEMOMENT  Aerodynamic moment in body axes.
%
%   FMB = computeMoment(c_moment, pdynmc, Sim)
%
%   Roll and yaw are scaled with the span, pitch with the mean chord.
%   Thrust is assumed to act through the centre of gravity and adds no moment.
%
%   Inputs
%     c_moment  [3x1]  Moment coefficients [Cl, Cm, Cn]
%     pdynmc    [1x1]  Dynamic pressure (Pa)
%     Sim       struct Vehicle geometry
%
%   Output
%     FMB       [3x1]  Aerodynamic moment in body axes [L, M, N] (N m)

refa = Sim.vehicle.geometry.refa;
refb = Sim.vehicle.geometry.refb;
refc = Sim.vehicle.geometry.refc;

FMB = pdynmc * refa * [refb; refc; refb] .* c_moment(:);

end

== matlab function GHAME_Public/GHAME Airframe/Kinematics/KINEMATICS/skew_sym ==
  data: x input; S output
function S = vec2skew(x)
% VEC2SKEW  Skew-symmetric matrix of a 3x1 vector.
%
%   S = vec2skew(x)
%
%   S*y equals cross(x, y) for any 3x1 vector y.
%
%   Input
%     x   [3x1]  Vector
%
%   Output
%     S   [3x3]  Skew-symmetric matrix

%   Author:    Thomas Harald Müller
%   GitHub:    https://github.com/ThomasHaraldMueller
%   Copyright: (c) 2026 Thomas Harald Müller, Hamburg, Germany
%   Free to use and modify, provided this notice is kept and the author is credited.

S = [  0    -x(3)   x(2);
      x(3)    0    -x(1);
     -x(2)   x(1)    0  ];

end

== matlab function GHAME_Public/GHAME Airframe/Kinematics/KINEMATICS/	Orthonormalizing TBI  ==
  data: TBI input; TBI output; ortho_error output
function [TBI, ortho_error] = normalizeT(TBI)
% NORMALIZET  First-order orthonormalization of a transformation matrix.
%
%   [TBI, ortho_error] = normalizeT(TBI)
%
%   Applies T <- T + 0.5*(I - T*T')*T, which removes the first-order
%   deviation from orthonormality. Repeated every step, this keeps the
%   integrated matrix close to a proper rotation.
%
%   Input
%     TBI          [3x3]  Integrated transformation matrix
%
%   Outputs
%     TBI          [3x3]  Corrected transformation matrix
%     ortho_error  [1x1]  Frobenius norm of (I - T*T') before correction,
%                         zero for an exactly orthonormal matrix

EE  = eye(3) - TBI * TBI';
TBI = TBI + 0.5 * EE * TBI;

% Includes off-diagonal terms, so non-perpendicular rows are detected too
ortho_error = norm(EE, 'fro');

end

== matlab function GHAME_Public/GHAME Airframe/Kinematics/KINEMATICS/Euler angles ==
  data: TBD input; psibdx output; thtbdx output; phibdx output; Sim parameter
function [psibdx, thtbdx, phibdx] = euler(TBD, Sim)
% EULER  Yaw, pitch and roll angles from the geodetic-to-body matrix.
%
%   [psibdx, thtbdx, phibdx] = euler(TBD, Sim)
%
%   Uses the 3-2-1 sequence (yaw, pitch, roll), so that
%   TBD(1,3) = -sin(theta), TBD(1,2)/TBD(1,1) = tan(psi) and
%   TBD(2,3)/TBD(3,3) = tan(phi). At theta = +-90 deg yaw and roll are not
%   separable (gimbal lock), and the split between them is arbitrary.
%
%   Inputs
%     TBD     [3x3]  Transformation matrix, geodetic to body
%     Sim     struct Constants (DEG)
%
%   Outputs (deg)
%     psibdx  Yaw angle (heading) in (-180, 180]
%     thtbdx  Pitch angle in [-90, 90]
%     phibdx  Roll angle in (-180, 180]

%   Author:    Thomas Harald Müller
%   GitHub:    https://github.com/ThomasHaraldMueller
%   Copyright: (c) 2026 Thomas Harald Müller, Hamburg, Germany
%   Free to use and modify, provided this notice is kept and the author is credited.

DEG = Sim.constants.DEG;

% Clamp guards against |TBD(1,3)| slightly above 1 from round-off
thtbd = asin(-max(min(TBD(1,3), 1), -1));
psibd = atan2(TBD(1,2), TBD(1,1));
phibd = atan2(TBD(2,3), TBD(3,3));

psibdx = DEG * psibd;
thtbdx = DEG * thtbd;
phibdx = DEG * phibd;

end

== matlab function GHAME_Public/GHAME Airframe/Kinematics/KINEMATICS/Aero angles ==
  data: VBAB input; alphax output; betax output; alppx output; phipx output; Sim parameter
function [alphax, betax, alppx, phipx] = angles_vbab(VBAB, Sim)
% ANGLES_VBAB  Aerodynamic angles from the air-relative velocity.
%
%   [alphax, betax, alppx, phipx] = angles_vbab(VBAB, Sim)
%
%   Inputs
%     VBAB    [3x1]  Air-relative velocity in body axes [u; v; w] (m/s)
%     Sim     struct Constants (DEG)
%
%   Outputs (deg)
%     alphax  Angle of attack
%     betax   Sideslip angle
%     alppx   Total angle of attack, between velocity and body x-axis
%     phipx   Aerodynamic roll angle in (-180, 180]
%
%   Undefined for zero airspeed.

%   Author:    Thomas Harald Müller
%   GitHub:    https://github.com/ThomasHaraldMueller
%   Copyright: (c) 2026 Thomas Harald Müller, Hamburg, Germany
%   Free to use and modify, provided this notice is kept and the author is credited.

DEG = Sim.constants.DEG;

u = VBAB(1);  v = VBAB(2);  w = VBAB(3);
V = norm(VBAB);

% Clamps guard against ratios slightly outside [-1, 1] from round-off
alpha = atan2(w, u);
beta  = asin(max(min(v / V, 1), -1));
alpp  = acos(max(min(u / V, 1), -1));
phip  = atan2(v, w);            % Also correct for v = 0 and v = w = 0

alphax = DEG * alpha;
betax  = DEG * beta;
alppx  = DEG * alpp;
phipx  = DEG * phip;

end
